simulink model "fft_one_input_test"  (Simulink 7.2)
settings: Solver=VariableStepDiscrete  StartTime=0.0  StopTime=64  RelTol=1e-3
libraries: xbsIndex_r4 x170, casper_library_misc x10, casper_library_delays x5, casper_library_reorder x2, casper_library_ffts_twiddle x1
(part 1 of 2)
settings Model: Creator=User  LastModifiedBy=root
settings OptimizationCC: InitFltsAndDblsToZero=on
settings DebuggingCC: SaveWithDisabledLinksMsg=none  SaveWithParameterizedLinksMsg=none

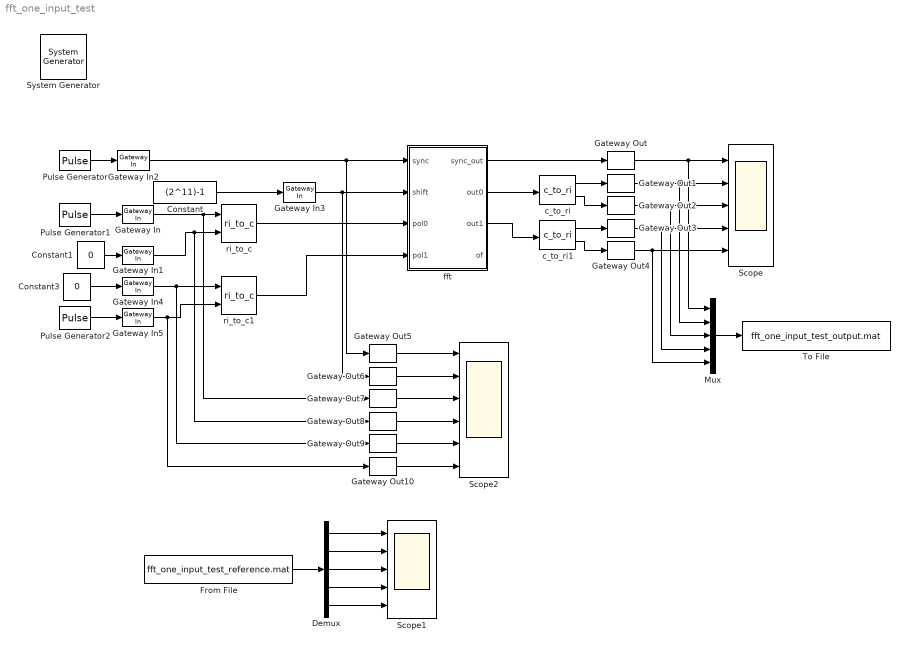
== system fft_one_input_test ==
  " System Generator" : xbsIndex_r4/ System Generator  Tag=genX  SystemSampleTime=-1  xilinxfamily=Virtex4  part=xc4vsx35  speed=-10  package=ff668  synthesis_tool=XST  clock_wrapper=Clock Enables  directory=./netlist  testbench=off  simulink_period=1  sysclk_period=100  dcm_input_clock_period=100  incr_netlist=off  trim_vbits=Everywhere in SubSystem  dbl_ovrd=According to Block Masks  core_generation=According to Block Masks  run_coregen=off  deprecated_control=off  eval_field=0  block_type=sysgen
      settings: block_version=10.1.1
  Constant : Constant  Value=(2^11)-1  OutDataType=sfix(16)  OutScaling=2^0
  Constant1 : Constant  Value=0  OutDataType=sfix(16)  OutScaling=2^0
  Constant3 : Constant  Value=0  OutDataType=sfix(16)  OutScaling=2^0
  Demux : Demux  Outputs=5
  From File : FromFile  FileName=fft_one_input_test_reference.mat  SampleTime=1
  Gateway In{,1,4..5} (4 alike) : xbsIndex_r4/Gateway In  arith_type="Signed  (2's comp)"  n_bits=8  bin_pt=7  quantization=Truncate  overflow=Wrap  period=1  dbl_ovrd=off  timing_constraint=None  locs_specified=off  LOCs={}  hdl_port=on  block_type=gatewayin
      settings: infoedit="Gateway in block.  Converts inputs of type Simulink integer, double and fixed point to  Xilinx fixed point type.<P><P>Hardware notes:  In hardware these blocks become top level input ports."  block_version=10.1.1
  Gateway In2 : xbsIndex_r4/Gateway In  arith_type=Boolean  n_bits=18  bin_pt=17  quantization=Truncate  overflow=Wrap  period=1  dbl_ovrd=off  timing_constraint=None  locs_specified=off  LOCs={}  hdl_port=on  block_type=gatewayin
      settings: infoedit="Gateway in block.  Converts inputs of type Simulink integer, double and fixed point to  Xilinx fixed point type.<P><P>Hardware notes:  In hardware these blocks become top level input ports."  block_version=10.1.1
  Gateway In3 : xbsIndex_r4/Gateway In  arith_type=Unsigned  n_bits=11  bin_pt=0  quantization=Truncate  overflow=Wrap  period=1  dbl_ovrd=off  timing_constraint=None  locs_specified=off  LOCs={}  hdl_port=on  block_type=gatewayin
      settings: infoedit="Gateway in block.  Converts inputs of type Simulink integer, double and fixed point to  Xilinx fixed point type.<P><P>Hardware notes:  In hardware these blocks become top level input ports."  block_version=10.1.1
  Gateway Out{,1..10} (11 alike) : xbsIndex_r4/Gateway Out  hdl_port=on  timing_constraint=None  locs_specified=off  LOCs={}  block_type=gatewayout
      settings: infoedit="Gateway out block.  Converts Xilinx fixed point inputs into ouputs of type Simulink integer, double, or fixed point.<P><P>Hardware notes:  In hardware these blocks become top level output ports or are discarded, depending on how they are configured."  block_version=10.1.1
  Mux : Mux  Inputs=5
  Pulse Generator : DiscretePulseGenerator  Period=2^4  PhaseDelay=11
  Pulse Generator1 : DiscretePulseGenerator  Period=2^2  PhaseDelay=13
  Pulse Generator2 : DiscretePulseGenerator  Period=2^3  PhaseDelay=13
  Scope : Scope  NumInputPorts=5
      settings: YMin=-1~0~0~-5~-5  YMax=2~1~1~5~5
  Scope1 : Scope  NumInputPorts=5
      settings: YMin=-1~0~0~-5~-5  YMax=2~1~1~5~5
  Scope2 : Scope  NumInputPorts=6
      settings: YMin=-1~0~0~-5~-5~-5  YMax=2~1~1~5~5~5  SaveName=ScopeData2
  To File : ToFile  Filename=fft_one_input_test_output.mat  MatrixName=output
  c_to_ri : casper_library_misc/c_to_ri  SystemSampleTime=-1  n_bits=8  bin_pt=7
      settings: AttributesFormatString=8_7 r/i
  c_to_ri1 : casper_library_misc/c_to_ri  SystemSampleTime=-1  n_bits=8  bin_pt=7
      settings: AttributesFormatString=8_7 r/i
  fft : Subsystem  AncestorBlock=casper_library_ffts/fft  mask(fft){FFTSize=2, input_bit_width=8, coeff_bit_width=8, n_inputs=0, quantization=Truncate, overflow=Saturate, add_latency=2, mult_latency=2, bram_latency=1, conv_latency=1, arch=Virtex5, opt_target=logic, coeffs_bit_limit=8, delays_bit_limit=8, specify_mult=off, mult_spec=[2                                      2], dsp48_adders=off}
      mask prompts: FFTSize "Size of FFT: (2^?)"; input_bit_width "Input/Output Bit Width"; coeff_bit_width "Coefficient Bit Width"; n_inputs "Number of Simultaneous Inputs: (2^?)"; quantization "Quantization Behavior"; overflow "Overflow Behavior"; add_latency "Add Latency"; mult_latency "Mult Latency"; bram_latency "BRAM Latency"; conv_latency "Convert latency"; arch "Architecture"; opt_target "Use less"; coeffs_bit_limit "Number bits above which to store stage's coefficients in BRAM (2^? bits)"; delays_bit_limit "Number bits above which to store stage's delays in BRAM (2^? bits)"; specify_mult "Specify multiplier use (behavioral HDL if not specified)"; mult_spec "Multiplier specification (0=core, 1=embedded, 2=behavioural) (left=1st stage)"; dsp48_adders "DSP48 adders in butterfly"
      mask init:
      | fft_init(gcb,...
      |     'FFTSize', FFTSize, ...
      |     'input_bit_width', input_bit_width, ...
      |     'coeff_bit_width', coeff_bit_width, ...
      |     'n_inputs', n_inputs, ...
      |     'quantization', quantization, ...
      |     'overflow', overflow, ...
      |     'add_latency', add_latency, ...
      |     'mult_latency', mult_latency, ...
      |     'bram_latency', bram_latency, ...
      |     'conv_latency', conv_latency, ...
      |     'arch', arch, ...
      |     'opt_target', opt_target, ...
      |     'coeffs_bit_limit', coeffs_bit_limit, ...
      |     'delays_bit_limit', delays_bit_limit, ...
      |     'specify_mult', specify_mult, ...
      |     'mult_spec', mult_spec, ...
      |     'dsp48_adders', dsp48_adders);
      settings: AttributesFormatString=|
      | 2 stages
      | (8,8)
      | Truncate
      | Saturate
      mask Help: eval('xlWeb(''http://casper.berkeley.edu/wiki/Fft'')')
      mask StyleString: edit,edit,edit,edit,popup(Truncate|Round  (unbiased: +/- Inf)|Round  (unbiased: Even Values)),popup(Wrap|Saturate|Error),edit,edit,edit,edit,popup(Virtex2Pro|Virtex5),popup(logic|multipliers),edit,edit,checkbox,edit,checkbox
      mask CallbackString:
      | % fft_size = eval(get_param(gcb, 'FFTSize'));
      | % old_vec = eval(get_param(gcb, 'mult_spec'));
      | 
      | % vec = 2.*ones(1,fft_size);
      | % old_size = length(old_vec);
      | 
      | % if(old_size <= fft_size), size = old_size;
      | % else, size = fft_size;
      | % end
      | 
      | % for n = 1:size, vec(n) = old_vec(n); end
      | % set_param(gcb, 'mult_spec', mat2str(vec));||||||||||fft_callback_arch(gcb);||||specify_mult = get_param(gcb,'specify_mult');
      | visibs = get_param(gcb, 'MaskVisibilities');
      | if( strcmp(specify_mult,'off')), visibs{16} = 'off';
      | else visibs{16} = 'on';
      | end
      | set_param(gcb, 'MaskVisibilities', visibs);
      | 
      | |% vec = eval( get_param(gcb, 'mult_spec'));
      | % vec_size = length(vec);
      | % fft_size = eval( get_param(gcb, 'FFTSize'));
      | % new_vec = 2.*ones(1, fft_size);
      | 
      | % if(vec_size <= fft_size), size = vec_size;
      | % else size = fft_size;
      | % end
      | 
      | % for n=1:size,
      | %    new_vec(n) = vec(n);
      | % end
      | % set_param(gcb, 'mult_spec', mat2str(new_vec));|fft_callback_dsp48_adders(gcb);
  ri_to_c : casper_library_misc/ri_to_c  SystemSampleTime=-1
  ri_to_c1 : casper_library_misc/ri_to_c  SystemSampleTime=-1
  wires:
  Pulse Generator/1 -> Gateway In2/1
  Gateway In2/1 -> Gateway Out5/1, fft/1(sync)
  Constant/1 -> Gateway In3/1
  Gateway In3/1 -> Gateway Out6/1, fft/2(shift)
  fft/1(sync_out) -> Gateway Out/1
  fft/2(out0) -> c_to_ri/1
  c_to_ri/1 -> Gateway Out1/1
  c_to_ri/2 -> Gateway Out2/1
  c_to_ri1/2 -> Gateway Out4/1
  c_to_ri1/1 -> Gateway Out3/1
  Gateway Out/1 -> Scope/1, Mux/1
  ri_to_c/1 -> fft/3(pol0)
  ri_to_c1/1 -> fft/4(pol1)
  Pulse Generator1/1 -> Gateway In/1
  Gateway In/1 -> ri_to_c/1, Gateway Out7/1
  Constant1/1 -> Gateway In1/1
  Gateway In1/1 -> ri_to_c/2, Gateway Out8/1
  Gateway In4/1 -> ri_to_c1/1, Gateway Out9/1
  Gateway In5/1 -> ri_to_c1/2, Gateway Out10/1
  Gateway Out1/1 -> Scope/2, Mux/2
  Gateway Out2/1 -> Scope/3, Mux/3
  Gateway Out3/1 -> Scope/4, Mux/4
  Gateway Out4/1 -> Scope/5, Mux/5
  Mux/1 -> To File/1
  From File/1 -> Demux/1
  Demux/1 -> Scope1/1
  Demux/2 -> Scope1/2
  Demux/3 -> Scope1/3
  Demux/4 -> Scope1/4
  Demux/5 -> Scope1/5
  Gateway Out5/1 -> Scope2/1
  Gateway Out6/1 -> Scope2/2
  Gateway Out7/1 -> Scope2/3
  Gateway Out8/1 -> Scope2/4
  Gateway Out9/1 -> Scope2/5
  Gateway Out10/1 -> Scope2/6
  Constant3/1 -> Gateway In4/1
  Pulse Generator2/1 -> Gateway In5/1
  fft/3(out1) -> c_to_ri1/1

== system fft_one_input_test/fft ==
  sync : Inport
  shift : Inport  Port=2
  pol0 : Inport  Port=3
  pol1 : Inport  Port=4
  fft_biplex0 : Subsystem  AncestorBlock=casper_library_ffts/fft_biplex  mask(fft_biplex){FFTSize=2, input_bit_width=8, coeff_bit_width=8, quantization=Truncate, overflow=Saturate, add_latency=2, mult_latency=2, bram_latency=1, conv_latency=1, arch=Virtex5, opt_target=logic, coeffs_bit_limit=8, delays_bit_limit=8, specify_mult=off, mult_spec=[2                                      2], dsp48_adders=off}
      mask prompts: FFTSize "Size of FFT: (2^? pnts)"; input_bit_width "Input/Output Bit Width"; coeff_bit_width "Coefficient Bit Width"; quantization "Quantization Behavior"; overflow "Overflow Behavior"; add_latency "Add Latency"; mult_latency "Mult Latency"; bram_latency "BRAM Latency"; conv_latency "Convert latency"; arch "Architecture"; opt_target "Use less"; coeffs_bit_limit "Number bits above which to store stage's coefficients in BRAM (2^? bits)"; delays_bit_limit "Number bits above which to implent stage's delays in BRAM (2^? bits)"; specify_mult "Specify multiplier use (behavioral HDL if not specified)"; mult_spec "Multiplier specification (0=core, 1=embedded, 2=behavioural) (left=1st stage)"; dsp48_adders "Use DSP48s for adders"
      mask init:
      | fft_biplex_init(gcb,...
      |     'FFTSize', FFTSize,...
      |     'input_bit_width', input_bit_width,...
      |     'coeff_bit_width', coeff_bit_width,...
      |     'quantization', quantization,...
      |     'overflow', overflow,...
      |     'add_latency', add_latency,...
      |     'mult_latency', mult_latency,...
      |     'bram_latency', bram_latency,...
      |     'conv_latency', conv_latency, ...
      |     'arch', arch, ...
      |     'opt_target', opt_target, ...
      |     'coeffs_bit_limit', coeffs_bit_limit, ...
      |     'delays_bit_limit', delays_bit_limit, ...
      |     'specify_mult', specify_mult,...
      |     'mult_spec', mult_spec, ...
      |     'dsp48_adders', dsp48_adders);
      settings: AttributesFormatString=|
      | 2 stages
      | Virtex5
      mask StyleString: edit,edit,edit,popup(Truncate|Round  (unbiased: +/- Inf)|Round  (unbiased: Even Values)),popup(Wrap|Saturate|Error),edit,edit,edit,edit,popup(Virtex2Pro|Virtex5),popup(logic|multipliers),edit,edit,checkbox,edit,checkbox
      mask CallbackString:
      | % fft_size = eval(get_param(gcb, 'FFTSize'));
      | % old_vec = eval(get_param(gcb, 'mult_spec'));
      | 
      | % vec = 2.*ones(1,fft_size);
      | % old_size = length(old_vec);
      | 
      | % if(old_size <= fft_size),
      | %    size = old_size;
      | % else,
      | %     size = fft_size;
      | % end
      | 
      | % for n = 1:size, vec(n) = old_vec(n); end
      | % set_param(gcb, 'mult_spec', mat2str(vec));|||||||||fft_callback_arch(gcb);||||specify_mult = get_param(gcb,'specify_mult');
      | visibs = get_param(gcb, 'MaskVisibilities');
      | 
      | if( strcmp(specify_mult,'off')), visibs{15} = 'off';
      | else, visibs{15} = 'on';
      | end
      | set_param(gcb, 'MaskVisibilities', visibs);
      | |% vec = eval( get_param(gcb, 'mult_spec'));
      | % vec_size = length(vec);
      | % fft_size = eval( get_param(gcb, 'FFTSize'));
      | % new_vec = 2.*ones(1, fft_size);
      | 
      | % if(vec_size <= fft_size), size = vec_size;
      | % else size = fft_size;
      | % end
      | 
      | % for n=1:size
      | %     new_vec(n) = vec(n);
      | % end
      | % set_param(gcb, 'mult_spec', mat2str(new_vec));|fft_callback_dsp48_adders(gcb);
  sync_out : Outport
  out0 : Outport  Port=2
  out1 : Outport  Port=3
  of : Outport  Port=4
  wires:
  pol0/1 -> fft_biplex0/1(pol1)
  pol1/1 -> fft_biplex0/2(pol2)
  shift/1 -> fft_biplex0/4(shift)
  sync/1 -> fft_biplex0/3(sync)
  fft_biplex0/1(pol1_out) -> out0/1
  fft_biplex0/2(pol2_out) -> out1/1
  fft_biplex0/4(sync_out) -> sync_out/1
  fft_biplex0/3(of) -> of/1

== system fft_one_input_test/fft/fft_biplex0 ==
  pol1 : Inport  OutDataType=sfix(16)  OutScaling=2^0
  pol2 : Inport  Port=2  OutDataType=sfix(16)  OutScaling=2^0
  sync : Inport  Port=3  OutDataType=sfix(16)  OutScaling=2^0
  shift : Inport  Port=4  OutDataType=sfix(16)  OutScaling=2^0
  biplex_core : Subsystem  AncestorBlock=casper_library_ffts/biplex_core  mask(biplex_core){FFTSize=2, input_bit_width=8, coeff_bit_width=8, quantization=Truncate, overflow=Saturate, add_latency=2, mult_latency=2, bram_latency=1, conv_latency=1, arch=Virtex5, opt_target=logic, coeffs_bit_limit=8, delays_bit_limit=8, specify_mult=off, mult_spec=[2                                      2], dsp48_adders=off}
      mask prompts: FFTSize "Size of FFT: (2^? pnts)"; input_bit_width "Input/Output Bit Width"; coeff_bit_width "Coefficient Bit Width"; quantization "Quantization Behavior"; overflow "Overflow Behavior"; add_latency "Add Latency"; mult_latency "Mult Latency"; bram_latency "BRAM Latency"; conv_latency "Convert latency"; arch "Architecture"; opt_target "Use less"; coeffs_bit_limit "Number bits above which to store stage's coefficients in BRAM (2^? bits)"; delays_bit_limit "Number bits above which to implent stage's delays in BRAM (2^? bits)"; specify_mult "Specify multiplier use (behavioural HDL if not specified)"; mult_spec "Multiplier specification (0=core, 1=embedded, 2=behavioural) (left=1st stage)"; dsp48_adders "Use DSP48s for adders"
      mask init:
      | biplex_core_init(gcb,...
      |     'FFTSize', FFTSize,...
      |     'input_bit_width', input_bit_width,...
      |     'coeff_bit_width', coeff_bit_width,...
      |     'quantization', quantization,...
      |     'overflow', overflow,...
      |     'add_latency', add_latency,...
      |     'mult_latency', mult_latency,...
      |     'bram_latency', bram_latency,...
      |     'conv_latency', conv_latency, ...
      |     'arch', arch, ...
      |     'opt_target', opt_target, ...
      |     'coeffs_bit_limit', coeffs_bit_limit, ...
      |     'delays_bit_limit', delays_bit_limit, ...
      |     'specify_mult', specify_mult, ...
      |     'mult_spec', mult_spec, ...
      |     'dsp48_adders', dsp48_adders );
      settings: AttributesFormatString=|
      | 2 stages
      | reduce logic
      | Virtex5
      mask StyleString: edit,edit,edit,popup(Truncate|Round  (unbiased: +/- Inf)|Round  (unbiased: Even Values)),popup(Wrap|Saturate|Error),edit,edit,edit,edit,popup(Virtex2Pro|Virtex5),popup(logic|multipliers),edit,edit,checkbox,edit,checkbox
      mask CallbackString:
      | % fft_size = eval(get_param(gcb, 'FFTSize'));
      | % old_vec = eval(get_param(gcb, 'mult_spec'));
      | 
      | % vec = 2.*ones(1,fft_size);
      | % old_size = length(old_vec);
      | 
      | % if(old_size <= fft_size),
      | %    size = old_size;
      | % else,
      | %     size = fft_size;
      | % end
      | 
      | % for n = 1:size, vec(n) = old_vec(n); end
      | % set_param(gcb, 'mult_spec', mat2str(vec));|||||||||fft_callback_arch(gcb);||||specify_mult = get_param(gcb,'specify_mult');
      | visibs = get_param(gcb,'MaskVisibilities');
      | if( strcmp(specify_mult,'off')), visibs{15} = 'off';
      | else, visibs{15} = 'on';
      | end
      | set_param(gcb, 'MaskVisibilities', visibs);
      | enables = get_param(gcb,'MaskVisibilities');
      | enables{15} = 'on';
      | set_param(gcb, 'MaskEnables', enables);
      | |% vec = eval( get_param(gcb, 'mult_spec'));
      | % vec_size = length(vec);
      | % fft_size = eval( get_param(gcb, 'FFTSize'));
      | % new_vec = 2.*ones(1, fft_size);
      | 
      | % if(vec_size <= fft_size), size = vec_size;
      | % else size = fft_size;
      | % end
      | 
      | % for n=1:size
      | %     new_vec(n) = vec(n);
      | % end
      | % set_param(gcb, 'mult_spec', mat2str(new_vec));|fft_callback_dsp48_adders(gcb);
  biplex_cplx_unscrambler : Subsystem  mask{FFTSize=2, bram_latency=1}
      mask prompts: FFTSize "Size of FFT: (2^? pnts)"; bram_latency "BRAM Latency"
      mask init:
      | blk = gcb;
      | if same_state(blk, 'FFTSize', FFTSize, 'bram_latency', bram_latency), return, end
      | map = bit_reverse(0:2^(FFTSize-1)-1, FFTSize-1);
      | set_param([blk,'/reorder'],'map',mat2str([map,map+2^(FFTSize-1)]));
      | set_param([blk,'/reorder'],'bram_latency', num2str(bram_latency));
      | set_param([blk,'/reorder1'],'map',mat2str([map+2^(FFTSize-1),map]));
      | set_param([blk,'/reorder1'],'bram_latency', num2str(bram_latency));
      | save_state(blk, 'FFTSize', FFTSize, 'bram_latency', bram_latency);
  pol1_out : Outport  OutDataType=sfix(16)  OutScaling=2^0
  pol2_out : Outport  Port=2  OutDataType=sfix(16)  OutScaling=2^0
  of : Outport  Port=3  OutDataType=sfix(16)  OutScaling=2^0
  sync_out : Outport  Port=4  OutDataType=sfix(16)  OutScaling=2^0
  wires:
  biplex_core/3(of) -> of/1
  biplex_cplx_unscrambler/1(pol1) -> pol1_out/1
  shift/1 -> biplex_core/4(shift)
  sync/1 -> biplex_core/3(sync)
  pol2/1 -> biplex_core/2(pol2)
  pol1/1 -> biplex_core/1(pol1)
  biplex_core/1(out1) -> biplex_cplx_unscrambler/1(even)
  biplex_core/2(out2) -> biplex_cplx_unscrambler/2(odd)
  biplex_core/4(sync_out) -> biplex_cplx_unscrambler/3(sync)
  biplex_cplx_unscrambler/2(pol2) -> pol2_out/1
  biplex_cplx_unscrambler/3(sync_out) -> sync_out/1

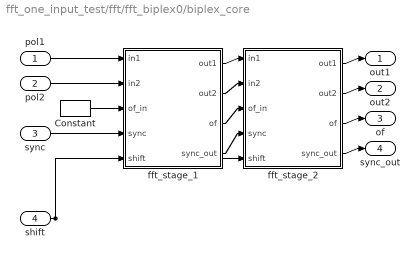
== system fft_one_input_test/fft/fft_biplex0/biplex_core ==
  pol1 : Inport
  pol2 : Inport  Port=2
  sync : Inport  Port=3
  shift : Inport  Port=4
  Constant : xbsIndex_r4/Constant  arith_type=Boolean  const=0  n_bits=16  bin_pt=14  explicit_period=off  period=1  equ=P=C  opselect=C  inp2=PCIN>>17  opr=+  inp1=P  carry=CIN  dbl_ovrd=off  block_type=constant
      settings: block_version=11.4
  fft_stage_1 : Subsystem  AncestorBlock=casper_library_ffts/fft_stage_n  mask(fft_stage_n){FFTSize=2, FFTStage=1, input_bit_width=8, coeff_bit_width=8, delays_bram=off, coeffs_bram=off, quantization=Truncate, overflow=Saturate, add_latency=2, mult_latency=2, bram_latency=1, conv_latency=1, arch=Virtex5, opt_target=logic, use_hdl=on, use_embedded=off, dsp48_adders=off}
      mask prompts: FFTSize "Size of FFT: (2^? pnts)"; FFTStage "Stage of FFT:"; input_bit_width "Input/Output Bit Width:"; coeff_bit_width "Coefficient Bit Width"; delays_bram "Implement Delays in BRAM:"; coeffs_bram "Store Coefficients in BRAM:"; quantization "Quantization Behavior"; overflow "Overflow Behavior"; add_latency "Add Latency"; mult_latency "Mult Latency"; bram_latency "BRAM Latency"; conv_latency "Convert latency"; arch "Architecture"; opt_target "Use less"; use_hdl "Use behavioural HDL for mutlipliers"; use_embedded "Use embedded multipliers"; dsp48_adders "Use DSP48s for adders"
      mask init:
      | fft_stage_n_init(gcb,...
      |     'FFTSize', FFTSize,...
      |     'FFTStage', FFTStage,...
      |     'input_bit_width', input_bit_width,...
      |     'coeff_bit_width', coeff_bit_width,...
      |     'delays_bram', delays_bram,...
      |     'coeffs_bram', coeffs_bram,...
      |     'quantization', quantization,...
      |     'overflow', overflow,...
      |     'add_latency', add_latency,...
      |     'mult_latency', mult_latency,...
      |     'bram_latency', bram_latency,...
      |     'conv_latency', conv_latency, ...
      |     'arch', arch, ...
      |     'opt_target', opt_target, ...
      |     'use_hdl', use_hdl,...
      |     'use_embedded', use_embedded, ...
      |     'dsp48_adders', dsp48_adders);
      settings: AttributesFormatString=|
      | [1/2]
      | delays in slices
      | coeffs in slices
      mask StyleString: edit,edit,edit,edit,checkbox,checkbox,popup(Truncate|Round  (unbiased: +/- Inf)|Round  (unbiased: Even Values)),popup(Wrap|Saturate|Error),edit,edit,edit,edit,popup(Virtex2Pro|Virtex5),popup(logic|multipliers),checkbox,checkbox,checkbox
      mask CallbackString:
      | ||||||||||||fft_callback_arch(gcb);||use_hdl = get_param(gcb,'use_hdl');
      | visibs = get_param(gcb, 'MaskVisibilities');
      | if( strcmp(use_hdl,'on')),
      |     visibs{16} = 'off';
      | else,
      |     visibs{16} = 'on';
      | end
      |     set_param(gcb, 'MaskVisibilities',visibs);||fft_callback_dsp48_adders(gcb);
  fft_stage_2 : Subsystem  AncestorBlock=casper_library_ffts/fft_stage_n  mask(fft_stage_n){FFTSize=2, FFTStage=2, input_bit_width=8, coeff_bit_width=8, delays_bram=off, coeffs_bram=off, quantization=Truncate, overflow=Saturate, add_latency=2, mult_latency=2, bram_latency=1, conv_latency=1, arch=Virtex5, opt_target=logic, use_hdl=on, use_embedded=off, dsp48_adders=off}
      mask prompts: FFTSize "Size of FFT: (2^? pnts)"; FFTStage "Stage of FFT:"; input_bit_width "Input/Output Bit Width:"; coeff_bit_width "Coefficient Bit Width"; delays_bram "Implement Delays in BRAM:"; coeffs_bram "Store Coefficients in BRAM:"; quantization "Quantization Behavior"; overflow "Overflow Behavior"; add_latency "Add Latency"; mult_latency "Mult Latency"; bram_latency "BRAM Latency"; conv_latency "Convert latency"; arch "Architecture"; opt_target "Use less"; use_hdl "Use behavioural HDL for mutlipliers"; use_embedded "Use embedded multipliers"; dsp48_adders "Use DSP48s for adders"
      mask init: same as fft_one_input_test/fft/fft_biplex0/biplex_core/fft_stage_1
      settings: AttributesFormatString=|
      | [2/2]
      | delays in slices
      | coeffs in slices
      mask StyleString: edit,edit,edit,edit,checkbox,checkbox,popup(Truncate|Round  (unbiased: +/- Inf)|Round  (unbiased: Even Values)),popup(Wrap|Saturate|Error),edit,edit,edit,edit,popup(Virtex2Pro|Virtex5),popup(logic|multipliers),checkbox,checkbox,checkbox
      mask CallbackString:
      | ||||||||||||fft_callback_arch(gcb);||use_hdl = get_param(gcb,'use_hdl');
      | visibs = get_param(gcb, 'MaskVisibilities');
      | if( strcmp(use_hdl,'on')),
      |     visibs{16} = 'off';
      | else,
      |     visibs{16} = 'on';
      | end
      |     set_param(gcb, 'MaskVisibilities',visibs);||fft_callback_dsp48_adders(gcb);
  out1 : Outport
  out2 : Outport  Port=2
  of : Outport  Port=3
  sync_out : Outport  Port=4
  wires:
  fft_stage_1/1(out1) -> fft_stage_2/1(in1)
  fft_stage_1/2(out2) -> fft_stage_2/2(in2)
  fft_stage_1/3(of) -> fft_stage_2/3(of_in)
  fft_stage_1/4(sync_out) -> fft_stage_2/4(sync)
  shift/1 -> fft_stage_2/5(shift), fft_stage_1/5(shift)
  pol1/1 -> fft_stage_1/1(in1)
  pol2/1 -> fft_stage_1/2(in2)
  Constant/1 -> fft_stage_1/3(of_in)
  sync/1 -> fft_stage_1/4(sync)
  fft_stage_2/1(out1) -> out1/1
  fft_stage_2/2(out2) -> out2/1
  fft_stage_2/3(of) -> of/1
  fft_stage_2/4(sync_out) -> sync_out/1

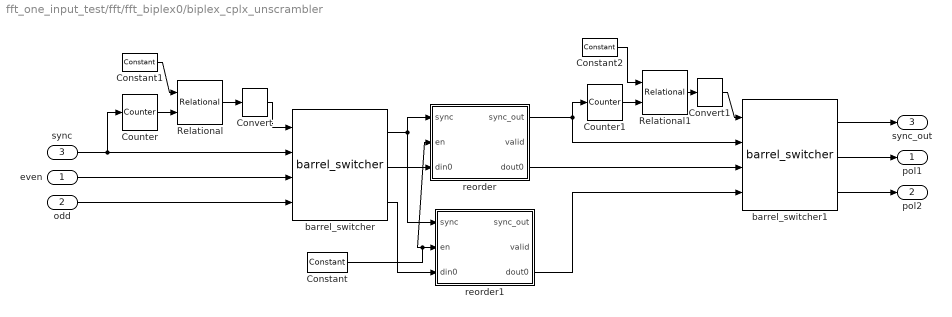
== system fft_one_input_test/fft/fft_biplex0/biplex_cplx_unscrambler ==
  even : Inport  OutDataType=sfix(16)  OutScaling=2^0
  odd : Inport  Port=2  OutDataType=sfix(16)  OutScaling=2^0
  sync : Inport  Port=3  OutDataType=sfix(16)  OutScaling=2^0
  Constant : xbsIndex_r4/Constant  arith_type=Boolean  const=1  n_bits=1  bin_pt=0  explicit_period=on  period=1  equ=P=C  opselect=C  inp2=PCIN>>17  opr=+  inp1=P  carry=CIN  dbl_ovrd=off  block_type=constant
      settings: block_version=9.1.01
  Constant1 : xbsIndex_r4/Constant  arith_type=Unsigned  const=2^(FFTSize-1)  n_bits=FFTSize  bin_pt=0  explicit_period=on  period=1  equ=P=C  opselect=C  inp2=PCIN>>17  opr=+  inp1=P  carry=CIN  dbl_ovrd=off  block_type=constant
      settings: block_version=9.1.01
  Constant2 : xbsIndex_r4/Constant  arith_type=Unsigned  const=2^(FFTSize-1)  n_bits=FFTSize  bin_pt=0  explicit_period=on  period=1  equ=P=C  opselect=C  inp2=PCIN>>17  opr=+  inp1=P  carry=CIN  dbl_ovrd=off  block_type=constant
      settings: block_version=9.1.01
  Convert : xbsIndex_r4/Convert  arith_type=Unsigned  n_bits=1  bin_pt=0  quantization=Truncate  overflow=Wrap  latency=0  dbl_ovrd=off  pipeline=off  block_type=convert
      settings: xl_area=[0, 0, 0, 0, 0, 0, 0]
  Convert1 : xbsIndex_r4/Convert  arith_type=Unsigned  n_bits=1  bin_pt=0  quantization=Truncate  overflow=Wrap  latency=0  dbl_ovrd=off  pipeline=off  block_type=convert
      settings: xl_area=[0, 0, 0, 0, 0, 0, 0]
  Counter : xbsIndex_r4/Counter  cnt_type=Free Running  cnt_to=Inf  operation=Up  start_count=0  cnt_by_val=1  arith_type=Unsigned  n_bits=FFTSize  bin_pt=0  load_pin=off  rst=on  en=off  explicit_period=off  period=1  dbl_ovrd=off  use_behavioral_HDL=off  implementation=Fabric  use_rpm=on  block_type=counter
      settings: xl_area=[0, 0, 0, 0, 0, 0, 0]  block_version=9.1.01
  Counter1 : xbsIndex_r4/Counter  cnt_type=Free Running  cnt_to=Inf  operation=Up  start_count=0  cnt_by_val=1  arith_type=Unsigned  n_bits=FFTSize  bin_pt=0  load_pin=off  rst=on  en=off  explicit_period=off  period=1  dbl_ovrd=off  use_behavioral_HDL=off  implementation=Fabric  use_rpm=on  block_type=counter
      settings: xl_area=[0, 0, 0, 0, 0, 0, 0]  block_version=9.1.01
  Relational : xbsIndex_r4/Relational  mode=a<=b  en=off  latency=0  dbl_ovrd=off  block_type=relational
      settings: xl_area=[0, 0, 0, 0, 0, 0, 0]  block_version=9.1.01
  Relational1 : xbsIndex_r4/Relational  mode=a<=b  en=off  latency=0  dbl_ovrd=off  block_type=relational
      settings: xl_area=[0, 0, 0, 0, 0, 0, 0]  block_version=9.1.01
  barrel_switcher : casper_library_reorder/barrel_switcher  SystemSampleTime=-1  n_inputs=1
      settings: AttributesFormatString=n_inputs=1
  barrel_switcher1 : casper_library_reorder/barrel_switcher  SystemSampleTime=-1  n_inputs=1
      settings: AttributesFormatString=n_inputs=1
  reorder : Subsystem  AncestorBlock=casper_library_reorder/reorder  mask(reorder){map=getfield( getfield( get_param( gcb,'UserData' ), 'parameters'),'map'), n_inputs=1, bram_latency=1, map_latency=0, double_buffer=0, bram_map=off}
      mask prompts: map "Output Order:"; n_inputs "Number of inputs"; bram_latency "BRAM Latency"; map_latency "Map Latency"; double_buffer "Double Buffer"; bram_map "Use BlockRAM for Map"
      mask init:
      | reorder_init(gcb, ...
      |     'map', map, ...
      |     'n_inputs', n_inputs, ...
      |     'bram_latency', bram_latency, ...
      |     'map_latency', map_latency, ...
      |     'double_buffer', double_buffer, ...
      |     'bram_map', bram_map);
      settings: AttributesFormatString=order=1
      mask Help: eval('xlWeb(''http://casper.berkeley.edu/wiki/Reorder'')')
  reorder1 : Subsystem  AncestorBlock=casper_library_reorder/reorder  mask(reorder){map=getfield( getfield( get_param( gcb,'UserData' ), 'parameters'),'map'), n_inputs=1, bram_latency=1, map_latency=0, double_buffer=0, bram_map=off}
      mask prompts: map "Output Order:"; n_inputs "Number of inputs"; bram_latency "BRAM Latency"; map_latency "Map Latency"; double_buffer "Double Buffer"; bram_map "Use BlockRAM for Map"
      mask init: same as fft_one_input_test/fft/fft_biplex0/biplex_cplx_unscrambler/reorder
      settings: AttributesFormatString=order=2
      mask Help: eval('xlWeb(''http://casper.berkeley.edu/wiki/Reorder'')')
  pol1 : Outport  OutDataType=sfix(16)  OutScaling=2^0
  pol2 : Outport  Port=2  OutDataType=sfix(16)  OutScaling=2^0
  sync_out : Outport  Port=3  OutDataType=sfix(16)  OutScaling=2^0
  wires:
  barrel_switcher/1 -> reorder/1(sync), reorder1/1(sync)
  barrel_switcher/2 -> reorder/3(din0)
  barrel_switcher/3 -> reorder1/3(din0)
  reorder/1(sync_out) -> barrel_switcher1/2, Counter1/1
  reorder/3(dout0) -> barrel_switcher1/3
  reorder1/3(dout0) -> barrel_switcher1/4
  even/1 -> barrel_switcher/3
  odd/1 -> barrel_switcher/4
  barrel_switcher1/1 -> sync_out/1
  barrel_switcher1/2 -> pol1/1
  barrel_switcher1/3 -> pol2/1
  sync/1 -> barrel_switcher/2, Counter/1
  Constant/1 -> reorder/2(en), reorder1/2(en)
  Constant1/1 -> Relational/1
  Counter/1 -> Relational/2
  Counter1/1 -> Relational1/2
  Constant2/1 -> Relational1/1
  Relational/1 -> Convert/1
  Relational1/1 -> Convert1/1
  Convert1/1 -> barrel_switcher1/1
  Convert/1 -> barrel_switcher/1

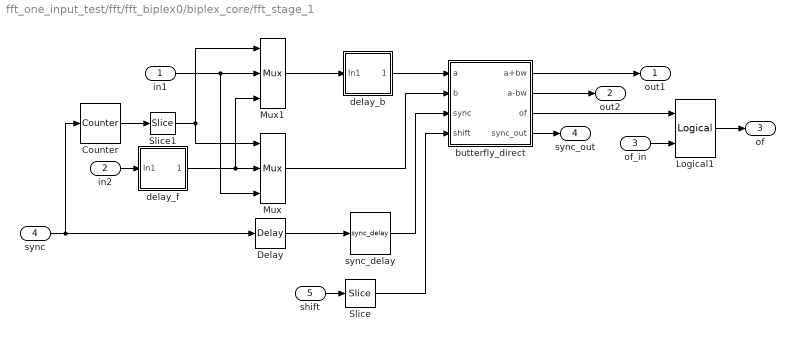
== system fft_one_input_test/fft/fft_biplex0/biplex_core/fft_stage_1 ==
  in1 : Inport  OutDataType=sfix(16)  OutScaling=2^0
  in2 : Inport  Port=2  OutDataType=sfix(16)  OutScaling=2^0
  of_in : Inport  Port=3  OutDataType=sfix(16)  OutScaling=2^0
  sync : Inport  Port=4  OutDataType=sfix(16)  OutScaling=2^0
  shift : Inport  Port=5  OutDataType=sfix(16)  OutScaling=2^0
  Counter : xbsIndex_r4/Counter  cnt_type=Free Running  cnt_to=Inf  operation=Up  start_count=0  cnt_by_val=1  arith_type=Unsigned  n_bits=FFTSize-FFTStage+1  bin_pt=0  load_pin=off  rst=on  en=off  explicit_period=off  period=1  dbl_ovrd=off  use_behavioral_HDL=off  implementation=Fabric  use_rpm=off  block_type=counter
      settings: xl_area=[0, 0, 0, 0, 0, 0, 0]  block_version=9.1.01
  Delay : xbsIndex_r4/Delay  en=off  latency=1  dbl_ovrd=off  reg_retiming=off  block_type=delay
      settings: xl_area=[0, 0, 0, 0, 0, 0, 0]  block_version=9.1.01
  Logical1 : xbsIndex_r4/Logical  logical_function=OR  inputs=2  en=off  latency=1  precision=Full  arith_type=Unsigned  n_bits=8  bin_pt=2  align_bp=on  dbl_ovrd=off  block_type=logical
      settings: xl_area=[0, 0, 0, 0, 0, 0, 0]  block_version=9.1.01
  Mux : xbsIndex_r4/Mux  inputs=2  en=off  latency=1  precision=Full  arith_type="Signed  (2's comp)"  n_bits=8  bin_pt=2  quantization=Truncate  overflow=Wrap  dbl_ovrd=off  block_type=mux
      settings: xl_area=[0, 0, 0, 0, 0, 0, 0]  block_version=9.1.01
  Mux1 : xbsIndex_r4/Mux  inputs=2  en=off  latency=1  precision=Full  arith_type="Signed  (2's comp)"  n_bits=8  bin_pt=2  quantization=Truncate  overflow=Wrap  dbl_ovrd=off  block_type=mux
      settings: xl_area=[0, 0, 0, 0, 0, 0, 0]  block_version=9.1.01
  Slice : xbsIndex_r4/Slice  nbits=1  boolean_output=on  mode=Lower Bit Location + Width  bit1=-(FFTStage - 1)  base1=MSB of Input  bit0=FFTStage - 1  base0=LSB of Input  dbl_ovrd=off  block_type=slice
      settings: infoedit="Extracts a given range of bits from each input sample and presents it at the output.  The output type is ordinarily unsigned with binary point at zero, but can be Boolean when the slice is one bit wide.<P><P>Hardware notes: In hardware this block costs nothing."  block_version=9.1.01
  Slice1 : xbsIndex_r4/Slice  nbits=1  boolean_output=off  mode=Upper Bit Location + Width  bit1=0  base1=MSB of Input  bit0=0  base0=LSB of Input  dbl_ovrd=off  block_type=slice
      settings: infoedit="Extracts a given range of bits from each input sample and presents it at the output.  The output type is ordinarily unsigned with binary point at zero, but can be Boolean when the slice is one bit wide.<P><P>Hardware notes: In hardware this block costs nothing."  block_version=9.1.01
  butterfly_direct : Subsystem  AncestorBlock=casper_library_ffts/butterfly_direct  mask(butterfly_direct){biplex=on, FFTSize=2, Coeffs=0, StepPeriod=1, coeffs_bram=off, coeff_bit_width=8, input_bit_width=8, bram_latency=1, add_latency=2, mult_latency=2, conv_latency=1, quantization=Truncate, overflow=Saturate, arch=Virtex5, opt_target=logic, use_hdl=on, use_embedded=off, dsp48_adders=off}
      mask prompts: biplex "Used in biplex FFT"; FFTSize "Size of FFT: (2^?)"; Coeffs "Coefficients: (0 to 2^(FFTSize-1)-1)"; StepPeriod "Coefficient Step Period: (2^?)"; coeffs_bram "Implement coefficients in BRAM"; coeff_bit_width "Coefficient Bit Width"; input_bit_width "Input/Output Bit Width:"; bram_latency "BRAM Latency"; add_latency "Add Latency"; mult_latency "Mult Latency"; conv_latency "Convert latency"; quantization "Quantization Behavior"; overflow "Overflow Behavior"; arch "Architecture"; opt_target "Use less"; use_hdl "Use behavioural HDL for multipliers"; use_embedded "Use embedded multipliers"; dsp48_adders "Use DSP48s for adders"
      mask init:
      | butterfly_direct_init(gcb,...
      |     'biplex', biplex,...
      |     'FFTSize', FFTSize,...
      |     'Coeffs', Coeffs,...
      |     'coeff_bit_width', coeff_bit_width,...
      |     'StepPeriod', StepPeriod,...
      |     'input_bit_width', input_bit_width,...
      |     'add_latency', add_latency,...
      |     'mult_latency', mult_latency,...
      |     'bram_latency', bram_latency,...
      |     'conv_latency', conv_latency, ...
      |     'coeffs_bram', coeffs_bram,...    
      |     'quantization', quantization,...
      |     'overflow', overflow,...
      |     'arch', arch,...
      |     'opt_target', opt_target,...
      |     'use_hdl', use_hdl,...
      |     'use_embedded', use_embedded,...
      |     'dsp48_adders', dsp48_adders);
      settings: AttributesFormatString=|
      | twiddle_pass_through
      | coeffs in slices
      mask StyleString: checkbox,edit,edit,edit,checkbox,edit,edit,edit,edit,edit,edit,popup(Truncate|Round  (unbiased: +/- Inf)|Round  (unbiased: Even Values)),popup(Wrap|Saturate|Error),popup(Virtex2Pro|Virtex5),popup(logic|multipliers),checkbox,checkbox,checkbox
      mask CallbackString:
      | ||%coeffs = eval(get_param(gcb,'Coeffs'));
      | %visibs = get_param(gcb,'MaskVisibilities');
      | %if length(coeffs) == 1,
      | %    visibs{4} = 'off'; visibs{5} = 'off';
      | %    visibs{6} = 'off';
      | %else
      | %    visibs{4} = 'on';
      | %    visibs{5} = 'on'; visibs{6} = 'on';
      | %end
      | %set_param(gcb, 'MaskVisibilities', visibs);|%coeffs = eval(get_param(gcb,'Coeffs'));
      | %visibs = get_param(gcb,'MaskVisibilities');
      | %if length(coeffs) == 1,
      | %    visibs{4} = 'off'; visibs{5} = 'off';
      | %    visibs{6} = 'off';
      | %else
      | %%    visibs{4} = 'on';
      | %    visibs{5} = 'on'; visibs{6} = 'on';
      | %end
      | %set_param(gcb, 'MaskVisibilities', visibs);|%coeffs = eval(get_param(gcb,'Coeffs'));
      | %visibs = get_param(gcb,'MaskVisibilities');
      | %if length(coeffs) == 1,
      | %    visibs{5} = 'off'; visibs{6} = 'off';
      | %    visibs{7} = 'off';
      | %else
      | %    visibs{5} = 'on';
      | %    visibs{6} = 'on'; visibs{7} = 'on';
      | %end
      | %set_param(gcb, 'MaskVisibilities', visibs);|||||||||fft_callback_arch(gcb);||use_hdl = get_param(gcb,'use_hdl');
      | visibs = get_param(gcb, 'MaskVisibilities');
      | if( strcmp(use_hdl,'on')),
      |     set_param(gcb, 'use_embedded','off');
      |     visibs{17} = 'off';
      | else,
      |     visibs{17} = 'on';
      | end
      |     set_param(gcb, 'MaskVisibilities',visibs);||fft_callback_dsp48_adders(gcb);
  delay_b : Subsystem  AncestorBlock=casper_library_delays/delay_slr  mask(delay_slr){DelayLen=2^(FFTSize-FFTStage)}
      mask prompts: DelayLen "Delay by:"
      mask help: A delay block that uses slices (SLR16s) for its storage.
      mask Help: eval('xlWeb(''http://casper.berkeley.edu/wiki/Delay_slr'')')
  delay_f : Subsystem  AncestorBlock=casper_library_delays/delay_slr  mask(delay_slr){DelayLen=2^(FFTSize-FFTStage)}
      mask prompts: DelayLen "Delay by:"
      mask help: A delay block that uses slices (SLR16s) for its storage.
      mask Help: eval('xlWeb(''http://casper.berkeley.edu/wiki/Delay_slr'')')
  sync_delay : casper_library_delays/sync_delay  SystemSampleTime=-1  DelayLen=2^(FFTSize - FFTStage)
  out1 : Outport  OutDataType=sfix(16)  OutScaling=2^0
  out2 : Outport  Port=2  OutDataType=sfix(16)  OutScaling=2^0
  of : Outport  Port=3  OutDataType=sfix(16)  OutScaling=2^0
  sync_out : Outport  Port=4  OutDataType=sfix(16)  OutScaling=2^0
  wires:
  shift/1 -> Slice/1
  of_in/1 -> Logical1/2
  Logical1/1 -> of/1
  Delay/1 -> sync_delay/1
  sync/1 -> Counter/1, Delay/1
  Counter/1 -> Slice1/1
  Mux/1 -> butterfly_direct/2(b)
  Mux1/1 -> delay_b/1(In1)
  delay_f/1(Out1) -> Mux1/3, Mux/2
  in1/1 -> Mux/3, Mux1/2
  Slice1/1 -> Mux/1, Mux1/1
  in2/1 -> delay_f/1(In1)
  delay_b/1(Out1) -> butterfly_direct/1(a)
  sync_delay/1 -> butterfly_direct/3(sync)
  Slice/1 -> butterfly_direct/4(shift)
  butterfly_direct/1(a+bw) -> out1/1
  butterfly_direct/2(a-bw) -> out2/1
  butterfly_direct/3(of) -> Logical1/1
  butterfly_direct/4(sync_out) -> sync_out/1

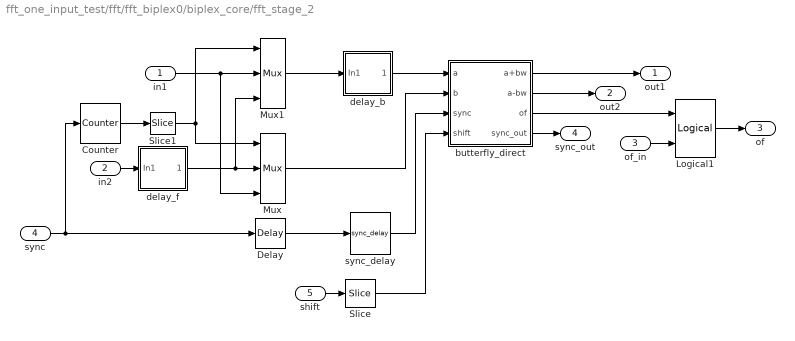
== system fft_one_input_test/fft/fft_biplex0/biplex_core/fft_stage_2 ==
  in1 : Inport  OutDataType=sfix(16)  OutScaling=2^0
  in2 : Inport  Port=2  OutDataType=sfix(16)  OutScaling=2^0
  of_in : Inport  Port=3  OutDataType=sfix(16)  OutScaling=2^0
  sync : Inport  Port=4  OutDataType=sfix(16)  OutScaling=2^0
  shift : Inport  Port=5  OutDataType=sfix(16)  OutScaling=2^0
  Counter : xbsIndex_r4/Counter  cnt_type=Free Running  cnt_to=Inf  operation=Up  start_count=0  cnt_by_val=1  arith_type=Unsigned  n_bits=FFTSize-FFTStage+1  bin_pt=0  load_pin=off  rst=on  en=off  explicit_period=off  period=1  dbl_ovrd=off  use_behavioral_HDL=off  implementation=Fabric  use_rpm=off  block_type=counter
      settings: xl_area=[0, 0, 0, 0, 0, 0, 0]  block_version=9.1.01
  Delay : xbsIndex_r4/Delay  en=off  latency=1  dbl_ovrd=off  reg_retiming=off  block_type=delay
      settings: xl_area=[0, 0, 0, 0, 0, 0, 0]  block_version=9.1.01
  Logical1 : xbsIndex_r4/Logical  logical_function=OR  inputs=2  en=off  latency=1  precision=Full  arith_type=Unsigned  n_bits=8  bin_pt=2  align_bp=on  dbl_ovrd=off  block_type=logical
      settings: xl_area=[0, 0, 0, 0, 0, 0, 0]  block_version=9.1.01
  Mux : xbsIndex_r4/Mux  inputs=2  en=off  latency=1  precision=Full  arith_type="Signed  (2's comp)"  n_bits=8  bin_pt=2  quantization=Truncate  overflow=Wrap  dbl_ovrd=off  block_type=mux
      settings: xl_area=[0, 0, 0, 0, 0, 0, 0]  block_version=9.1.01
  Mux1 : xbsIndex_r4/Mux  inputs=2  en=off  latency=1  precision=Full  arith_type="Signed  (2's comp)"  n_bits=8  bin_pt=2  quantization=Truncate  overflow=Wrap  dbl_ovrd=off  block_type=mux
      settings: xl_area=[0, 0, 0, 0, 0, 0, 0]  block_version=9.1.01
  Slice : xbsIndex_r4/Slice  nbits=1  boolean_output=on  mode=Lower Bit Location + Width  bit1=-(FFTStage - 1)  base1=MSB of Input  bit0=FFTStage - 1  base0=LSB of Input  dbl_ovrd=off  block_type=slice
      settings: infoedit="Extracts a given range of bits from each input sample and presents it at the output.  The output type is ordinarily unsigned with binary point at zero, but can be Boolean when the slice is one bit wide.<P><P>Hardware notes: In hardware this block costs nothing."  block_version=9.1.01
  Slice1 : xbsIndex_r4/Slice  nbits=1  boolean_output=off  mode=Upper Bit Location + Width  bit1=0  base1=MSB of Input  bit0=0  base0=LSB of Input  dbl_ovrd=off  block_type=slice
      settings: infoedit="Extracts a given range of bits from each input sample and presents it at the output.  The output type is ordinarily unsigned with binary point at zero, but can be Boolean when the slice is one bit wide.<P><P>Hardware notes: In hardware this block costs nothing."  block_version=9.1.01
  butterfly_direct : Subsystem  AncestorBlock=casper_library_ffts/butterfly_direct  mask(butterfly_direct){biplex=on, FFTSize=2, Coeffs=[0                                      1], StepPeriod=0, coeffs_bram=off, coeff_bit_width=8, input_bit_width=8, bram_latency=1, add_latency=2, mult_latency=2, conv_latency=1, quantization=Truncate, overflow=Saturate, arch=Virtex5, opt_target=logic, use_hdl=on, use_embedded=off, dsp48_adders=off}
      mask prompts: biplex "Used in biplex FFT"; FFTSize "Size of FFT: (2^?)"; Coeffs "Coefficients: (0 to 2^(FFTSize-1)-1)"; StepPeriod "Coefficient Step Period: (2^?)"; coeffs_bram "Implement coefficients in BRAM"; coeff_bit_width "Coefficient Bit Width"; input_bit_width "Input/Output Bit Width:"; bram_latency "BRAM Latency"; add_latency "Add Latency"; mult_latency "Mult Latency"; conv_latency "Convert latency"; quantization "Quantization Behavior"; overflow "Overflow Behavior"; arch "Architecture"; opt_target "Use less"; use_hdl "Use behavioural HDL for multipliers"; use_embedded "Use embedded multipliers"; dsp48_adders "Use DSP48s for adders"
      mask init: same as fft_one_input_test/fft/fft_biplex0/biplex_core/fft_stage_1/butterfly_direct
      settings: AttributesFormatString=|
      | twiddle_stage_2
      | coeffs in slices
      mask StyleString: checkbox,edit,edit,edit,checkbox,edit,edit,edit,edit,edit,edit,popup(Truncate|Round  (unbiased: +/- Inf)|Round  (unbiased: Even Values)),popup(Wrap|Saturate|Error),popup(Virtex2Pro|Virtex5),popup(logic|multipliers),checkbox,checkbox,checkbox
      mask CallbackString:
      | ||%coeffs = eval(get_param(gcb,'Coeffs'));
      | %visibs = get_param(gcb,'MaskVisibilities');
      | %if length(coeffs) == 1,
      | %    visibs{4} = 'off'; visibs{5} = 'off';
      | %    visibs{6} = 'off';
      | %else
      | %    visibs{4} = 'on';
      | %    visibs{5} = 'on'; visibs{6} = 'on';
      | %end
      | %set_param(gcb, 'MaskVisibilities', visibs);|%coeffs = eval(get_param(gcb,'Coeffs'));
      | %visibs = get_param(gcb,'MaskVisibilities');
      | %if length(coeffs) == 1,
      | %    visibs{4} = 'off'; visibs{5} = 'off';
      | %    visibs{6} = 'off';
      | %else
      | %%    visibs{4} = 'on';
      | %    visibs{5} = 'on'; visibs{6} = 'on';
      | %end
      | %set_param(gcb, 'MaskVisibilities', visibs);|%coeffs = eval(get_param(gcb,'Coeffs'));
      | %visibs = get_param(gcb,'MaskVisibilities');
      | %if length(coeffs) == 1,
      | %    visibs{5} = 'off'; visibs{6} = 'off';
      | %    visibs{7} = 'off';
      | %else
      | %    visibs{5} = 'on';
      | %    visibs{6} = 'on'; visibs{7} = 'on';
      | %end
      | %set_param(gcb, 'MaskVisibilities', visibs);|||||||||fft_callback_arch(gcb);||use_hdl = get_param(gcb,'use_hdl');
      | visibs = get_param(gcb, 'MaskVisibilities');
      | if( strcmp(use_hdl,'on')),
      |     set_param(gcb, 'use_embedded','off');
      |     visibs{17} = 'off';
      | else,
      |     visibs{17} = 'on';
      | end
      |     set_param(gcb, 'MaskVisibilities',visibs);||fft_callback_dsp48_adders(gcb);
  delay_b : Subsystem  AncestorBlock=casper_library_delays/delay_slr  mask(delay_slr){DelayLen=2^(FFTSize-FFTStage)}
      mask prompts: DelayLen "Delay by:"
      mask help: A delay block that uses slices (SLR16s) for its storage.
      mask Help: eval('xlWeb(''http://casper.berkeley.edu/wiki/Delay_slr'')')
  delay_f : Subsystem  AncestorBlock=casper_library_delays/delay_slr  mask(delay_slr){DelayLen=2^(FFTSize-FFTStage)}
      mask prompts: DelayLen "Delay by:"
      mask help: A delay block that uses slices (SLR16s) for its storage.
      mask Help: eval('xlWeb(''http://casper.berkeley.edu/wiki/Delay_slr'')')
  sync_delay : casper_library_delays/sync_delay  SystemSampleTime=-1  DelayLen=2^(FFTSize - FFTStage)
  out1 : Outport  OutDataType=sfix(16)  OutScaling=2^0
  out2 : Outport  Port=2  OutDataType=sfix(16)  OutScaling=2^0
  of : Outport  Port=3  OutDataType=sfix(16)  OutScaling=2^0
  sync_out : Outport  Port=4  OutDataType=sfix(16)  OutScaling=2^0
  wires:
  shift/1 -> Slice/1
  of_in/1 -> Logical1/2
  Logical1/1 -> of/1
  Delay/1 -> sync_delay/1
  sync/1 -> Counter/1, Delay/1
  Counter/1 -> Slice1/1
  Mux/1 -> butterfly_direct/2(b)
  Mux1/1 -> delay_b/1(In1)
  delay_f/1(Out1) -> Mux1/3, Mux/2
  in1/1 -> Mux/3, Mux1/2
  Slice1/1 -> Mux/1, Mux1/1
  in2/1 -> delay_f/1(In1)
  delay_b/1(Out1) -> butterfly_direct/1(a)
  sync_delay/1 -> butterfly_direct/3(sync)
  Slice/1 -> butterfly_direct/4(shift)
  butterfly_direct/1(a+bw) -> out1/1
  butterfly_direct/2(a-bw) -> out2/1
  butterfly_direct/3(of) -> Logical1/1
  butterfly_direct/4(sync_out) -> sync_out/1

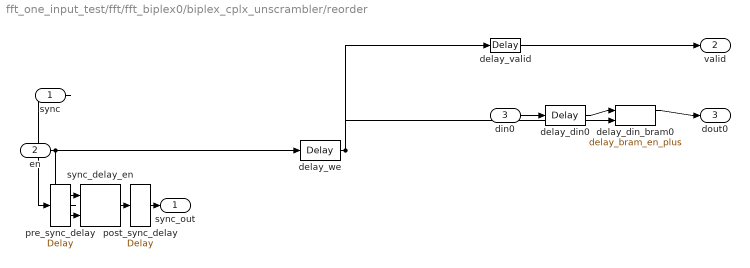
== system fft_one_input_test/fft/fft_biplex0/biplex_cplx_unscrambler/reorder ==
  sync : Inport  OutDataType=sfix(16)  OutScaling=2^0
  en : Inport  Port=2  OutDataType=sfix(16)  OutScaling=2^0
  din0 : Inport  Port=3  OutDataType=sfix(16)  OutScaling=2^0
  delay_din0 : xbsIndex_r4/Delay  en=off  latency=1  dbl_ovrd=off  reg_retiming=off  block_type=delay
      settings: xl_area=[0, 0, 0, 0, 0, 0, 0]  block_version=9.1.01
  delay_din_bram0 : casper_library_delays/delay_bram_en_plus  SystemSampleTime=-1  DelayLen=length(map)  bram_latency=bram_latency
  delay_valid : xbsIndex_r4/Delay  en=off  latency=2  dbl_ovrd=off  reg_retiming=off  block_type=delay
      settings: xl_area=[0, 0, 0, 0, 0, 0, 0]  block_version=9.1.01
  delay_we : xbsIndex_r4/Delay  en=off  latency=0  dbl_ovrd=off  reg_retiming=off  block_type=delay
      settings: xl_area=[0, 0, 0, 0, 0, 0, 0]  block_version=9.1.01
  post_sync_delay : xbsIndex_r4/Delay  en=off  latency=2  dbl_ovrd=off  reg_retiming=off  block_type=delay
      settings: xl_area=[0, 0, 0, 0, 0, 0, 0]  block_version=9.1.01
  pre_sync_delay : xbsIndex_r4/Delay  en=off  latency=0  dbl_ovrd=off  reg_retiming=off  block_type=delay
      settings: xl_area=[0, 0, 0, 0, 0, 0, 0]  block_version=9.1.01
  sync_delay_en : casper_library_delays/sync_delay_en  SystemSampleTime=-1  DelayLen=4
  sync_out : Outport  OutDataType=sfix(16)  OutScaling=2^0
  valid : Outport  Port=2  OutDataType=sfix(16)  OutScaling=2^0
  dout0 : Outport  Port=3  OutDataType=sfix(16)  OutScaling=2^0
  wires:
  sync/1 -> pre_sync_delay/1
  pre_sync_delay/1 -> sync_delay_en/1
  sync_delay_en/1 -> post_sync_delay/1
  en/1 -> sync_delay_en/2, delay_we/1
  post_sync_delay/1 -> sync_out/1
  delay_we/1 -> delay_valid/1, delay_din_bram0/2
  delay_valid/1 -> valid/1
  din0/1 -> delay_din0/1
  delay_din0/1 -> delay_din_bram0/1
  delay_din_bram0/1 -> dout0/1
